simulink model "HeartSim"  (R2024b)
settings: Solver=FixedStepAuto  StartTime=0.0  StopTime=inf  FixedStep=0.01  RelTol=1e-3
model workspace (MAT data in the model file):
  BPM = 60
  sample_time = 1e-06
undefined symbols (not defined in the file): daq
libraries: daqlib x3
settings Model: Creator=cbusc  LastModifiedBy=cbusc

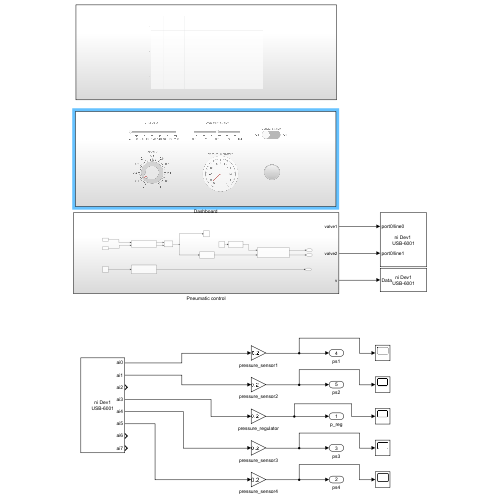
[thumbnail: Simulink's stored preview of the top-level diagram]
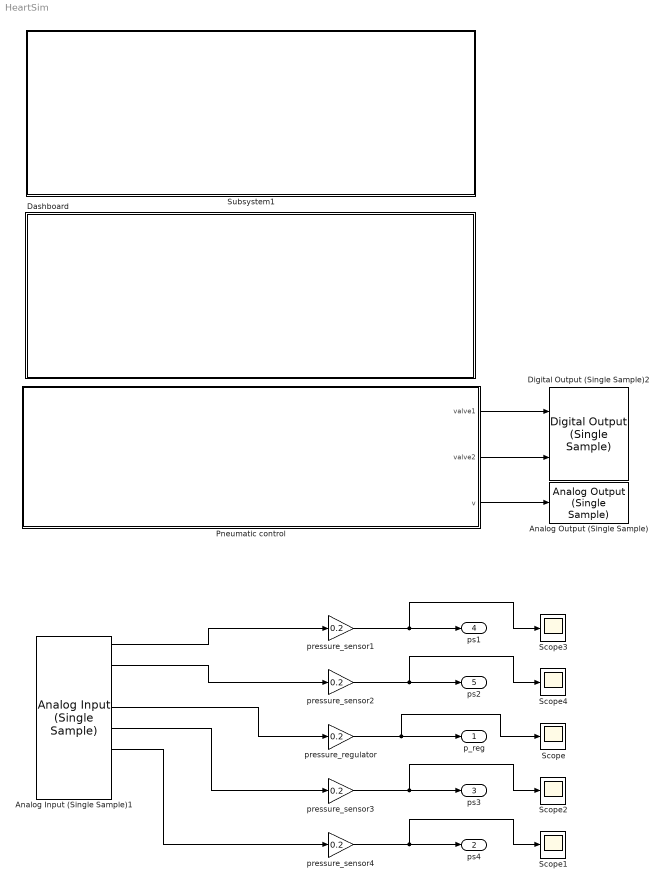
== system HeartSim ==
  Analog Input (Single Sample)1 : daqlib/Analog Input (Single Sample)  DeviceMenu=ni Dev1 (USB-6001)  Device=ni Dev1 (USB-6001)  ObjConstructor=daq.createSession('ni')  BlockSampleTime=0.1  NChannelsSelected=8  Channels=1$ai0$$Dev1$1$1$1$1$#1$ai1$$Dev1$1$1$1$1$#1$ai2$$Dev1$1$1$1$1$#1$ai3$$Dev1$1$1$1$1$#1$ai4$$Dev1$1$1$1$1$#1$ai5$$Dev1$1$1$1$1$#1$ai6$$Dev1$1$1$1$1$#1$ai7$$Dev1$1$1$1$1$#  NPorts=1 per channel  OutputTimestamp=off
  Analog Output (Single Sample) : daqlib/Analog Output (Single Sample)  DeviceMenu=ni Dev1 (USB-6001)  Device=ni Dev1 (USB-6001)  ObjConstructor=daq.createSession('ni')  NChannelsSelected=1  Channels=1$ao0$$Dev1$1$1$N/A$#0$ao1$$Dev1$1$1$N/A$#  NPorts=1 for all channels  BlockSampleTime=0.01
  Dashboard : Subsystem
  Digital Output (Single Sample)2 : daqlib/Digital Output (Single Sample)  DeviceMenu=ni Dev1 (USB-6001)  Device=ni Dev1 (USB-6001)  ObjConstructor=daq.createSession('ni')  BlockSampleTime=0.01  IsDigitalInput=off  NLinesSelected=2  Lines=1$port0/line0$$Dev1$#1$port0/line1$$Dev1$#0$port0/line2$$Dev1$#0$port0/line3$$Dev1$#0$port0/line4$$Dev1$#0$port0/line5$$Dev1$#0$port0/line6$$Dev1$#0$port0/line7$$Dev1$#0$port1/line0$$Dev1$#0$port1/line1$$Dev1$#0$port1/line2$$Dev1$#0$port1/line3$$Dev1$#0$port2/line0$$Dev1$#  NPorts=1 per line
  Pneumatic control : Subsystem
  Scope{,1..4} (5 alike) : Scope
  Subsystem1 : Subsystem
  pressure_regulator : Gain  Gain=0.2
  pressure_sensor{1..4} (4 alike) : Gain  Gain=0.2
  p_reg : Outport
  ps4 : Outport  Port=2
  ps3 : Outport  Port=3
  ps1 : Outport  Port=4
  ps2 : Outport  Port=5
  wires:
  Pneumatic control/1(valve1) -> Digital Output (Single Sample)2/1
  Pneumatic control/2(valve2) -> Digital Output (Single Sample)2/2
  Pneumatic control/3(v) -> Analog Output (Single Sample)/1
  pressure_regulator/1 -> p_reg/1, Scope/1
  Analog Input (Single Sample)1/4 -> pressure_regulator/1
  pressure_sensor4/1 -> Scope1/1, ps4/1
  Analog Input (Single Sample)1/6 -> pressure_sensor4/1
  pressure_sensor3/1 -> Scope2/1, ps3/1
  Analog Input (Single Sample)1/5 -> pressure_sensor3/1
  pressure_sensor1/1 -> Scope3/1, ps1/1
  Analog Input (Single Sample)1/1 -> pressure_sensor1/1
  pressure_sensor2/1 -> Scope4/1, ps2/1
  Analog Input (Single Sample)1/2 -> pressure_sensor2/1

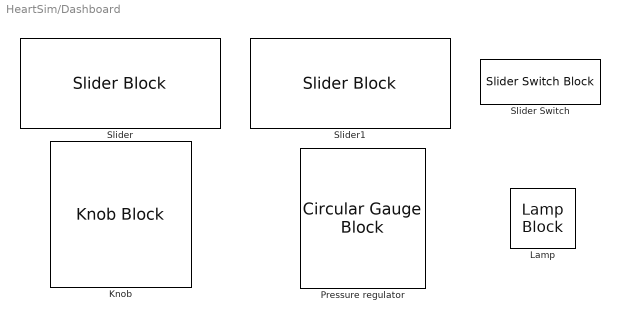
== system HeartSim/Dashboard ==
  Knob : KnobBlock  ScaleMax=1  TickInterval=0.1
  Lamp : LampBlock  LabelPosition=Hide
  Pressure regulator : CircularGaugeBlock  ScaleMax=2
  Slider : SliderBlock  ScaleMin=40  ScaleMax=200
  Slider Switch : SliderSwitchBlock
      settings: Values={{'Off', 'On'}, [0 1]}
  Slider1 : SliderBlock  ScaleMin=0.2  ScaleMax=0.4  TickInterval=0.05

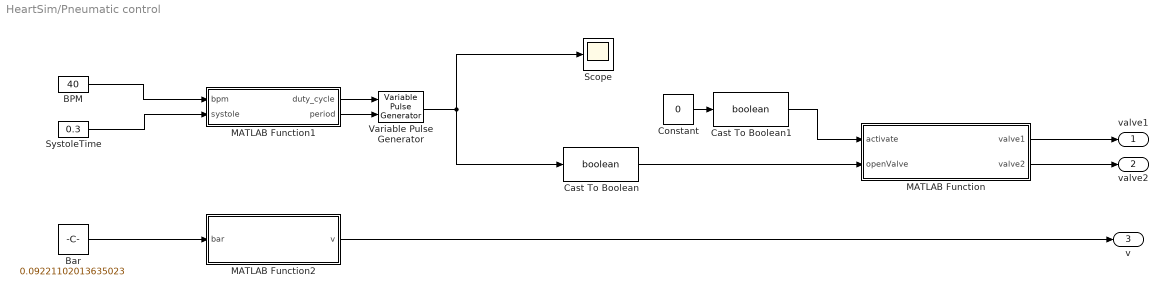
== system HeartSim/Pneumatic control ==
  BPM : Constant  Value=40
  Bar : Constant  Value=0.09221102013635023
  Cast To Boolean : DataTypeConversion  OutDataTypeStr=boolean  SaturateOnIntegerOverflow=off  RndMeth=Floor
  Cast To Boolean1 : DataTypeConversion  OutDataTypeStr=boolean  SaturateOnIntegerOverflow=off  RndMeth=Floor
  Constant : Constant  Value=0
  MATLAB Function : MATLAB Function  TreatAsAtomicUnit=on
  MATLAB Function1 : MATLAB Function  TreatAsAtomicUnit=on
  MATLAB Function2 : MATLAB Function  TreatAsAtomicUnit=on
  Scope : Scope
  SystoleTime : Constant  Value=0.3
  Variable Pulse Generator : VariablePulseGenerator  RunAtFixedTimeIntervals=on  SampleTime=0.01
  valve1 : Outport
  valve2 : Outport  Port=2
  v : Outport  Port=3
  wires:
  Bar/1 -> MATLAB Function2/1(bar)
  MATLAB Function1/2(period) -> Variable Pulse Generator/2
  Variable Pulse Generator/1 -> Scope/1, Cast To Boolean/1
  Cast To Boolean/1 -> MATLAB Function/2(openValve)
  BPM/1 -> MATLAB Function1/1(bpm)
  MATLAB Function/1(valve1) -> valve1/1
  Constant/1 -> Cast To Boolean1/1
  MATLAB Function1/1(duty_cycle) -> Variable Pulse Generator/1
  SystoleTime/1 -> MATLAB Function1/2(systole)
  Cast To Boolean1/1 -> MATLAB Function/1(activate)
  MATLAB Function2/1(v) -> v/1
  MATLAB Function/2(valve2) -> valve2/1

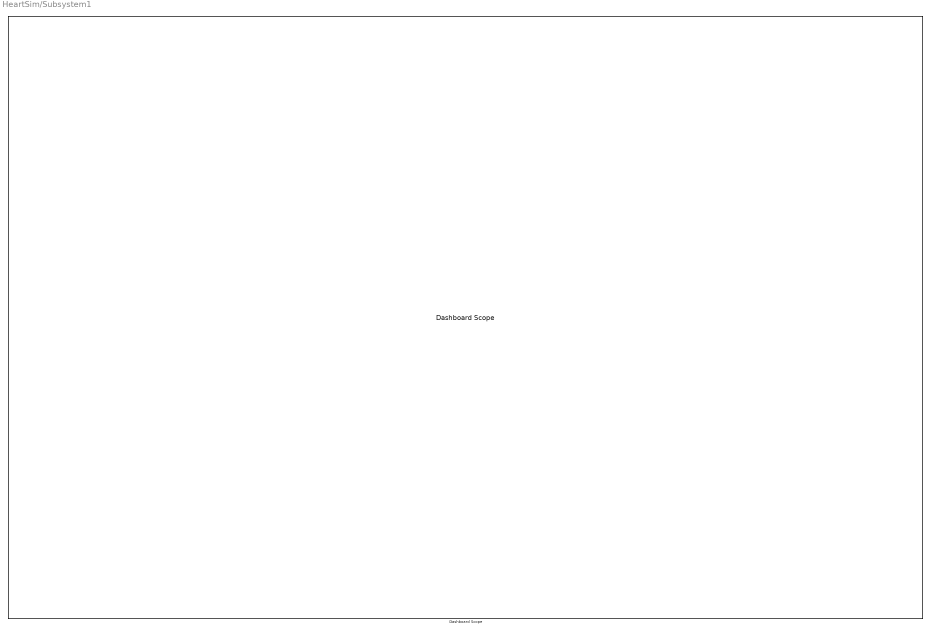
== system HeartSim/Subsystem1 ==
  Dashboard Scope : DashboardScope

== matlab function HeartSim/Pneumatic control/MATLAB Function1 ==
  data: duty_cycle output; bpm input; period output; systole input
function [duty_cycle, period] = f(bpm, systole)
% bpm in beats per minute
% systole in seconds

period = 60 / bpm;
duty_cycle = (systole / period);

== matlab function HeartSim/Pneumatic control/MATLAB Function ==
  data: activate input; valve1 output; openValve input; valve2 output
function [valve1, valve2] = controlValves(activate, openValve)
% controlValves - returns inverse logic for two valves
%
% Inputs:
%   openValve1 - boolean or binary input (1 = open, 0 = closed)
%
% Outputs:
%   valve1 - state of valve 1
%   valve2 - state of valve 2 (inverse of valve 1)

if activate
    valve1 = openValve;
    valve2 = ~valve1;
else 
    valve1 = openValve;
    valve2 = openValve;
end

== matlab function HeartSim/Pneumatic control/MATLAB Function2 ==
  data: bar input; v output
function v = barToVoltage(bar)
% barToVoltage - Converts pressure in bar to voltage (0–10 V)
% Assumes linear mapping: 0 bar → 0 V, 2 bar → 10 V

    % Check limits
    if bar < 0
        warning('Input below 0 bar. Clipping to 0.');
        bar = 0;
    elseif bar > 2
        warning('Input above 2 bar. Clipping to 2.');
        bar = 2;
    end

    % Linear mapping
    v = (bar / 2) * 10;
end
